simulink model "drive_fb_unpack"  (R2026b)
settings: Solver=VariableStepAuto
undefined symbols (not defined in the file or in its folder): P
libraries: simulink x3, svdutilitieslib x3
settings Model: Creator=aomar  LastModifiedBy=aomar

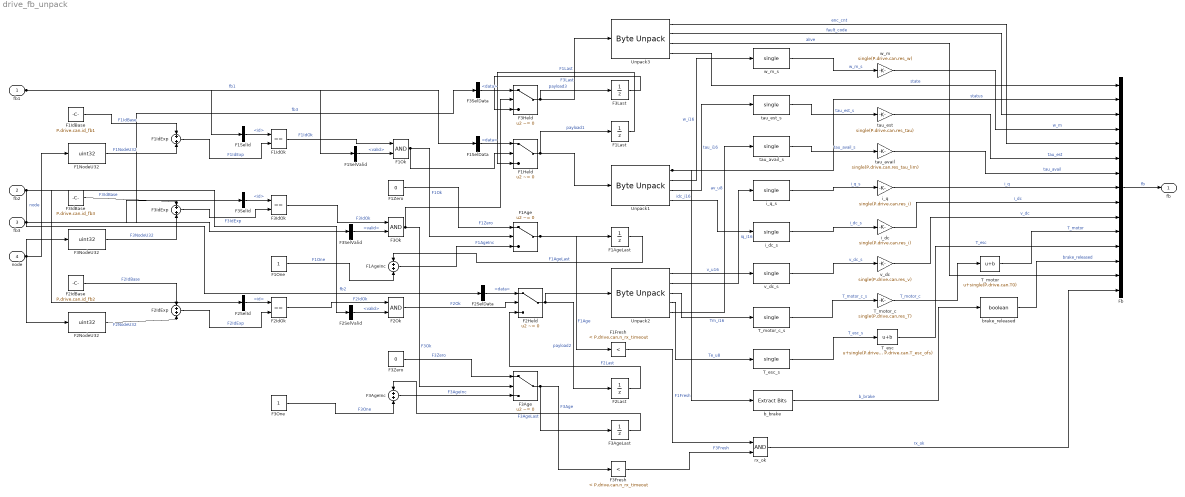
== system drive_fb_unpack ==
  fb1 : Inport  OutDataTypeStr=Bus: Bus_CanFrame8
  fb2 : Inport  Port=2  OutDataTypeStr=Bus: Bus_CanFrame8
  fb3 : Inport  Port=3  OutDataTypeStr=Bus: Bus_CanFrame8
  node : Inport  Port=4  OutDataTypeStr=uint8
  F1Age : Switch  Criteria=u2 ~= 0  SaturateOnIntegerOverflow=off  InputSameDT=off
  F1AgeInc : Sum  OutDataTypeStr=uint8  SaturateOnIntegerOverflow=on
  F1AgeLast : UnitDelay  InitialCondition=P.drive.can.n_rx_timeout  SampleTime=-1
  F1Fresh : simulink/Logic and Bit Operations/Compare To Constant  relop=<  const=P.drive.can.n_rx_timeout  OutDataTypeStr=boolean
  F1Held : Switch  Criteria=u2 ~= 0  SaturateOnIntegerOverflow=off  InputSameDT=off
  F1IdBase : Constant  Value=P.drive.can.id_fb1  OutDataTypeStr=uint32
  F1IdExp : Sum  OutDataTypeStr=uint32  SaturateOnIntegerOverflow=on
  F1IdOk : RelationalOperator  Operator===  OutDataTypeStr=boolean  RndMeth=Simplest  InputSameDT=off
  F1Last : UnitDelay  InitialCondition=zeros(8,1)  SampleTime=-1
  F1NodeU32 : DataTypeConversion  OutDataTypeStr=uint32  RndMeth=Nearest
  F1Ok : Logic  AllPortsSameDT=off  OutDataTypeStr=boolean
  F1One : Constant  OutDataTypeStr=uint8
  F1SelData : BusSelector  OutputSignals=data
  F1SelId : BusSelector  OutputSignals=id
  F1SelValid : BusSelector  OutputSignals=valid
  F1Zero : Constant  Value=0  OutDataTypeStr=uint8
  F2Held : Switch  Criteria=u2 ~= 0  SaturateOnIntegerOverflow=off  InputSameDT=off
  F2IdBase : Constant  Value=P.drive.can.id_fb2  OutDataTypeStr=uint32
  F2IdExp : Sum  OutDataTypeStr=uint32  SaturateOnIntegerOverflow=on
  F2IdOk : RelationalOperator  Operator===  OutDataTypeStr=boolean  RndMeth=Simplest  InputSameDT=off
  F2Last : UnitDelay  InitialCondition=zeros(8,1)  SampleTime=-1
  F2NodeU32 : DataTypeConversion  OutDataTypeStr=uint32  RndMeth=Nearest
  F2Ok : Logic  AllPortsSameDT=off  OutDataTypeStr=boolean
  F2SelData : BusSelector  OutputSignals=data
  F2SelId : BusSelector  OutputSignals=id
  F2SelValid : BusSelector  OutputSignals=valid
  F3Age : Switch  Criteria=u2 ~= 0  SaturateOnIntegerOverflow=off  InputSameDT=off
  F3AgeInc : Sum  OutDataTypeStr=uint8  SaturateOnIntegerOverflow=on
  F3AgeLast : UnitDelay  InitialCondition=P.drive.can.n_rx_timeout  SampleTime=-1
  F3Fresh : simulink/Logic and Bit Operations/Compare To Constant  relop=<  const=P.drive.can.n_rx_timeout  OutDataTypeStr=boolean
  F3Held : Switch  Criteria=u2 ~= 0  SaturateOnIntegerOverflow=off  InputSameDT=off
  F3IdBase : Constant  Value=P.drive.can.id_fb3  OutDataTypeStr=uint32
  F3IdExp : Sum  OutDataTypeStr=uint32  SaturateOnIntegerOverflow=on
  F3IdOk : RelationalOperator  Operator===  OutDataTypeStr=boolean  RndMeth=Simplest  InputSameDT=off
  F3Last : UnitDelay  InitialCondition=zeros(8,1)  SampleTime=-1
  F3NodeU32 : DataTypeConversion  OutDataTypeStr=uint32  RndMeth=Nearest
  F3Ok : Logic  AllPortsSameDT=off  OutDataTypeStr=boolean
  F3One : Constant  OutDataTypeStr=uint8
  F3SelData : BusSelector  OutputSignals=data
  F3SelId : BusSelector  OutputSignals=id
  F3SelValid : BusSelector  OutputSignals=valid
  F3Zero : Constant  Value=0  OutDataTypeStr=uint8
  Fb : BusCreator  Inputs=15  OutDataTypeStr=Bus: Bus_DriveSideFb  NonVirtualBus=on
  T_esc : Bias  Bias=single(P.drive.can.T0 - P.drive.can.T_esc_ofs)  SaturateOnIntegerOverflow=off
  T_esc_s : DataTypeConversion  OutDataTypeStr=single  RndMeth=Nearest
  T_motor : Bias  Bias=single(P.drive.can.T0)  SaturateOnIntegerOverflow=off
  T_motor_c : Gain  Gain=single(P.drive.can.res_T)  ParamDataTypeStr=single  OutDataTypeStr=single
  T_motor_c_s : DataTypeConversion  OutDataTypeStr=single  RndMeth=Nearest
  Unpack1 : svdutilitieslib/Byte Unpack  dimensions={1,1,1,1}  datatypes={'uint16','int16','int16','int16'}  byteAlign=1  blockPlatform=arduinoert
      settings: LibrarySourceBlock=mcblib/Signal Management/Byte Unpack
  Unpack2 : svdutilitieslib/Byte Unpack  dimensions={1,1,1,1,1}  datatypes={'uint16','int16','int16','uint8','uint8'}  byteAlign=1  blockPlatform=arduinoert
      settings: LibrarySourceBlock=mcblib/Signal Management/Byte Unpack
  Unpack3 : svdutilitieslib/Byte Unpack  dimensions={1,1,1,1}  datatypes={'int32','uint16','uint8','uint8'}  byteAlign=1  blockPlatform=arduinoert
      settings: LibrarySourceBlock=mcblib/Signal Management/Byte Unpack
  b_brake : simulink/Logic and Bit Operations/Extract Bits  bitsToExtract=Range of bits  numBits=8  bitIdxRange=[4 4]  outScalingMode=Treat bit field as an integer
  brake_released : DataTypeConversion  OutDataTypeStr=boolean  RndMeth=Nearest
  i_dc : Gain  Gain=single(P.drive.can.res_i)  ParamDataTypeStr=single  OutDataTypeStr=single
  i_dc_s : DataTypeConversion  OutDataTypeStr=single  RndMeth=Nearest
  i_q : Gain  Gain=single(P.drive.can.res_i)  ParamDataTypeStr=single  OutDataTypeStr=single
  i_q_s : DataTypeConversion  OutDataTypeStr=single  RndMeth=Nearest
  rx_ok : Logic  AllPortsSameDT=off  OutDataTypeStr=boolean
  tau_avail : Gain  Gain=single(P.drive.can.res_tau_lim)  ParamDataTypeStr=single  OutDataTypeStr=single
  tau_avail_s : DataTypeConversion  OutDataTypeStr=single  RndMeth=Nearest
  tau_est : Gain  Gain=single(P.drive.can.res_tau)  ParamDataTypeStr=single  OutDataTypeStr=single
  tau_est_s : DataTypeConversion  OutDataTypeStr=single  RndMeth=Nearest
  v_dc : Gain  Gain=single(P.drive.can.res_v)  ParamDataTypeStr=single  OutDataTypeStr=single
  v_dc_s : DataTypeConversion  OutDataTypeStr=single  RndMeth=Nearest
  w_m : Gain  Gain=single(P.drive.can.res_w)  ParamDataTypeStr=single  OutDataTypeStr=single
  w_m_s : DataTypeConversion  OutDataTypeStr=single  RndMeth=Nearest
  fb : Outport  OutDataTypeStr=Bus: Bus_DriveSideFb
  wires:
  fb1/1 -> F1SelValid/1, F1SelData/1, F1SelId/1  "fb1"
  fb3/1 -> F3SelData/1, F3SelId/1, F3SelValid/1  "fb3"
  F1IdBase/1 -> F1IdExp/1  "F1IdBase"
  F3IdBase/1 -> F3IdExp/1  "F3IdBase"
  F2IdBase/1 -> F2IdExp/1  "F2IdBase"
  F1NodeU32/1 -> F1IdExp/2  "F1NodeU32"
  F3NodeU32/1 -> F3IdExp/2  "F3NodeU32"
  F2NodeU32/1 -> F2IdExp/2  "F2NodeU32"
  F1IdExp/1 -> F1IdOk/2  "F1IdExp"
  F3IdExp/1 -> F3IdOk/2  "F3IdExp"
  F2IdExp/1 -> F2IdOk/2  "F2IdExp"
  F1SelId/1 -> F1IdOk/1  "<id>"
  F3SelId/1 -> F3IdOk/1  "<id>"
  F2SelId/1 -> F2IdOk/1  "<id>"
  F1IdOk/1 -> F1Ok/1  "F1IdOk"
  F3IdOk/1 -> F3Ok/1  "F3IdOk"
  F1One/1 -> F1AgeInc/2  "F1One"
  F2IdOk/1 -> F2Ok/1  "F2IdOk"
  F3One/1 -> F3AgeInc/2  "F3One"
  F3SelValid/1 -> F3Ok/2  "<valid>"
  F2SelValid/1 -> F2Ok/2  "<valid>"
  F1SelValid/1 -> F1Ok/2  "<valid>"
  F1AgeInc/1 -> F1Age/3  "F1AgeInc"
  F3AgeInc/1 -> F3Age/3  "F3AgeInc"
  F1Zero/1 -> F1Age/1  "F1Zero"
  F3Ok/1 -> F3Age/2, F3Held/2  "F3Ok"
  F2Ok/1 -> F2Held/2  "F2Ok"
  F3Zero/1 -> F3Age/1  "F3Zero"
  F1Ok/1 -> F1Age/2, F1Held/2  "F1Ok"
  F3SelData/1 -> F3Held/1  "<data>"
  F1SelData/1 -> F1Held/1  "<data>"
  F2SelData/1 -> F2Held/1  "<data>"
  F3Held/1 -> Unpack3/1, F3Last/1  "payload3"
  F1Held/1 -> Unpack1/1, F1Last/1  "payload1"
  F1Age/1 -> F1Fresh/1, F1AgeLast/1  "F1Age"
  F3Age/1 -> F3Fresh/1, F3AgeLast/1  "F3Age"
  F2Held/1 -> F2Last/1, Unpack2/1  "payload2"
  F1Fresh/1 -> rx_ok/1  "F1Fresh"
  F3Fresh/1 -> rx_ok/2  "F3Fresh"
  F3Last/1 -> F3Held/3  "F3Last"
  F1Last/1 -> F1Held/3  "F1Last"
  F1AgeLast/1 -> F1AgeInc/1  "F1AgeLast"
  F2Last/1 -> F2Held/3  "F2Last"
  F3AgeLast/1 -> F3AgeInc/1  "F3AgeLast"
  Unpack3/1 -> Fb/5  "enc_cnt"
  Unpack3/2 -> Fb/3  "fault_code"
  Unpack3/3 -> Fb/14  "alive"
  Unpack3/4 -> Fb/1  "state"
  Unpack1/1 -> b_brake/1, Fb/2  "status"
  Unpack1/2 -> w_m_s/1  "w_i16"
  Unpack1/3 -> tau_est_s/1  "tau_i16"
  Unpack1/4 -> i_dc_s/1  "idc_i16"
  Unpack2/1 -> v_dc_s/1  "v_u16"
  Unpack2/2 -> i_q_s/1  "iq_i16"
  Unpack2/3 -> T_motor_c_s/1  "Tm_i16"
  Unpack2/4 -> T_esc_s/1  "Te_u8"
  Unpack2/5 -> tau_avail_s/1  "av_u8"
  rx_ok/1 -> Fb/15  "rx_ok"
  w_m_s/1 -> w_m/1  "w_m_s"
  tau_est_s/1 -> tau_est/1  "tau_est_s"
  tau_avail_s/1 -> tau_avail/1  "tau_avail_s"
  i_q_s/1 -> i_q/1  "i_q_s"
  i_dc_s/1 -> i_dc/1  "i_dc_s"
  v_dc_s/1 -> v_dc/1  "v_dc_s"
  T_motor_c_s/1 -> T_motor_c/1  "T_motor_c_s"
  T_esc_s/1 -> T_esc/1  "T_esc_s"
  b_brake/1 -> brake_released/1  "b_brake"
  w_m/1 -> Fb/4  "w_m"
  tau_est/1 -> Fb/6  "tau_est"
  tau_avail/1 -> Fb/7  "tau_avail"
  i_q/1 -> Fb/8  "i_q"
  i_dc/1 -> Fb/9  "i_dc"
  v_dc/1 -> Fb/10  "v_dc"
  T_motor_c/1 -> T_motor/1  "T_motor_c"
  T_esc/1 -> Fb/12  "T_esc"
  T_motor/1 -> Fb/11  "T_motor"
  brake_released/1 -> Fb/13  "brake_released"
  Fb/1 -> fb/1  "fb"
  fb2/1 -> F2SelValid/1, F2SelId/1, F2SelData/1  "fb2"
  node/1 -> F1NodeU32/1, F2NodeU32/1, F3NodeU32/1  "node"
